simulink model "ECO_RM_WEC_SD_PI"  (R2025a)
settings: Solver=ode4  StartTime=0  StopTime=120  FixedStep=0.00025  MaxStep=0.00025  RelTol=1e-3
values from neighbouring files (symbols this model uses):
  s = tf('s')    [Compensated_loop_analysis.m]    (also in Plant_analysis.m)
  simu = simulationClass()    [wecSimInputFile.m]
  Z = (B + Bv)      + 1i*(omega0*(M + A) - C/omega0)    [Reference_velocity_calculation.m]
undefined symbols (not defined in the file or in its folder): body, constraint, geometry, hydroData, pto, X, Y
libraries: nesl_utility x9, sm_lib x5, WECSim_Lib_Body_Elements x2, WECSim_Lib_Frames x1, slpidlib x1, WECSim_Lib_Constraints x1
settings Model: Creator=pam1061  LastModifiedBy=Viki Vagnerova
settings SolverCC: ZeroCrossControl=DisableAll  AutoInsertRateTranBlk=on
settings DataIOCC: ReturnWorkspaceOutputs=off
settings OptimizationCC: SimCompilerOptimization=on

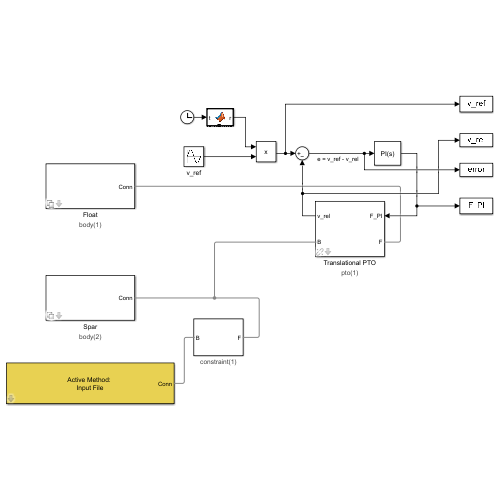
[thumbnail: Simulink's stored preview of the top-level diagram]
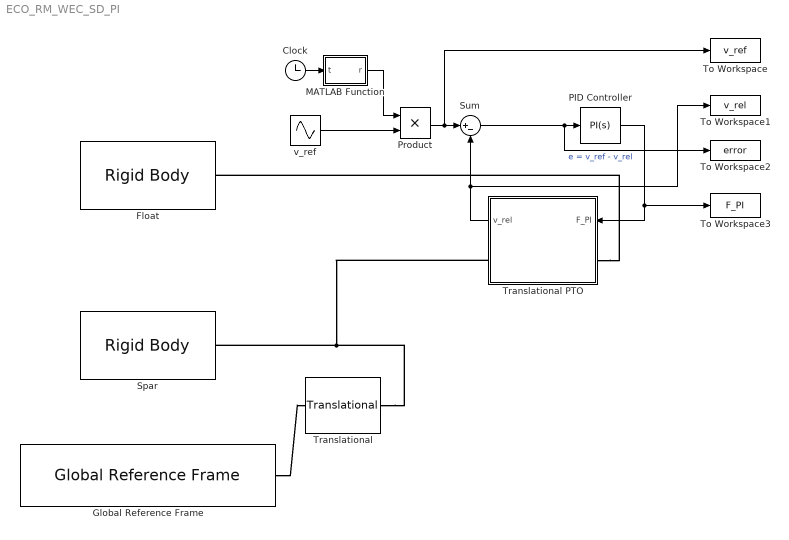
== system ECO_RM_WEC_SD_PI ==
  Clock : Clock
  Float : WECSim_Lib_Body_Elements/Rigid Body  body=body(1)  h5File=hydroData/*.h5  geometryFile=geometry/*.stl  mass=0  inertia=0 0 0  inertiaProducts=0 0 0  nonHydro=0  nonlinearHydro=0  centerGravity=0 0 0  centerBuoyancy=0 0 0  dof=6  volume=0  displacement=0 0 0  axis=0 1 0  angle=0  option=0  cd=0 0 0  ca=0 0 0  area=0 0 0  VME=0  rgME=0 0 0  z=0 0 1
  Global Reference Frame : WECSim_Lib_Frames/Global Reference Frame  waves=waves  simu=simu  InputMethod=Input File  InputFile=wecSimInputFile.m  mode=normal  explorer=off  solver=ode4  startTime=0  rampTime=100  endTime=400  dt=0.1  cicEndTime=60  stateSpace=0  WaveClass=regular  height=2.5  period=8  elevationFile=NOT DEFINED  spectrumFile=NOT DEFINED  direction=0  spread=1  spectrumType=NOT DEFINED  phaseSeed=0  option=EqualEnergy
  MATLAB Function : MATLAB Function  TreatAsAtomicUnit=on
  PID Controller : slpidlib/PID Controller  Controller=PI  Form=Parallel  TimeDomain=Continuous-time  UseExternalTs=off  SampleTime=-1  IntegratorMethod=Forward Euler  FilterMethod=Forward Euler  ControllerParametersSource=internal  P=1625.088066  I=4991.194750  UseKiTs=off  D=0  UseExternalDerivativeSource=off  N=100  UseFilter=on  TunerSelectOption=Transfer Function Based (PID Tuner App)  InitialConditionSource=internal  InitialConditionForIntegrator=0  InitialConditionForFilter=0  DifferentiatorICPrevScaledInput=0  ExternalReset=none  TrackingMode=off  Kt=1  LimitOutput=off  SatLimitsSource=internal  UpperSaturationLimit=inf  LowerSaturationLimit=-inf  LinearizeAsGain=on  AntiWindupMode=none  Kb=1  LimitIntegrator=off  UpperIntegratorSaturationLimit=inf  LowerIntegratorSaturationLimit=-inf  POutMin=[]  POutMax=[]  IOutMin=[]  IOutMax=[]  DOutMin=[]  DOutMax=[]  NOutMin=[]  NOutMax=[]  SumOutMin=[]  SumOutMax=[]  SaturationOutMin=[]  SaturationOutMax=[]  PParamMin=[]  PParamMax=[]  IParamMin=[]  IParamMax=[]  DParamMin=[]  DParamMax=[]  NParamMin=[]  NParamMax=[]  KbParamMin=[]  KbParamMax=[]  KtParamMin=[]  KtParamMax=[]  KbOutMin=[]  KbOutMax=[]  KtOutMin=[]  KtOutMax=[]  IntegratorOutMin=[]  IntegratorOutMax=[]  FilterOutMin=[]  FilterOutMax=[]  SumI1OutMin=[]  SumI1OutMax=[]  SumI2OutMin=[]  SumI2OutMax=[]  SumI3OutMin=[]  SumI3OutMax=[]  SumI4OutMin=[]  SumI4OutMax=[]  SumDOutMin=[]  SumDOutMax=[]  DifferentiatorOutMin=[]  DifferentiatorOutMax=[]  FilterDiffOutCoefMin=[]  FilterDiffOutCoefMax=[]  ReciprocalOutMin=[]  ReciprocalOutMax=[]  SumDenOutMin=[]  SumDenOutMax=[]  SumNumOutMin=[]  SumNumOutMax=[]  DivideOutMin=[]  DivideOutMax=[]  UdiffTsProdOutMin=[]  UdiffTsProdOutMax=[]  NTsProdOutMin=[]  NTsProdOutMax=[]  UintegralTsProdOutMin=[]  UintegralTsProdOutMax=[]  UngainTsProdOutMin=[]  UngainTsProdOutMax=[]  ClampingZeroOutDataTypeStr=Inherit: Inherit via back propagation  ClampingZeroOutMin=[]  ClampingZeroOutMax=[]  FilterDenConstantOutDataTypeStr=Inherit: Inherit via back propagation  FilterDenConstantOutMin=[]  FilterDenConstantOutMax=[]  PCopyOutDataTypeStr=Inherit: Inherit via back propagation  PCopyOutMin=[]  PCopyOutMax=[]  NCopyOutDataTypeStr=Inherit: Inherit via back propagation  NCopyOutMin=[]  NCopyOutMax=[]  IntegratorContinuousStateAttributes=''  IntegratorStateMustResolveToSignalObject=off  IntegratorRTWStateStorageClass=Auto  FilterContinuousStateAttributes=''  FilterStateMustResolveToSignalObject=off  FilterRTWStateStorageClass=Auto  ParallelPVariant=InternalParameters  IdealPVariant=Disabled  IVariant=InternalParameters  DVariant=Disabled  IntegratorVariant=Continuous  SatVariant=Disabled  AWVariant=Passthrough  PCopyVariant=Disabled  TRVariant=Disabled  FdbkBlocksVariant=Forward  IdealPFdbkVariant=Disabled  SatFdbkVariant=Disabled  DerivativeFilterVariant=Disabled  NVariant=Disabled  NCopyVariant=Disabled_SignalSpec  FilterICVariant=Disabled  IntegratorICVariant=InternalICs  ExternalResetVariant=Disabled  TRSumVariant=Passthrough  SumFdbkVariant=Disabled  SumVariant=Sum_PI  TsampFilterVariant=InternalTs  TsampNgainVariant=Passthrough  TsampIntegralVariant=Disabled_SignalSpec  ExternalSaturationOutDataTypeStr=Inherit: Same as second input  DerivativeSourceVariant=Disabled  PreIntVariant=InternalPreInt
  Product : Product
  Spar : WECSim_Lib_Body_Elements/Rigid Body  body=body(2)  h5File=hydroData/*.h5  geometryFile=geometry/*.stl  mass=0  inertia=0 0 0  inertiaProducts=0 0 0  nonHydro=0  nonlinearHydro=0  centerGravity=0 0 0  centerBuoyancy=0 0 0  dof=6  volume=0  displacement=0 0 0  axis=0 1 0  angle=0  option=0  cd=0 0 0  ca=0 0 0  area=0 0 0  VME=0  rgME=0 0 0  z=0 0 1
  Sum : Sum  Inputs=|+-
  To Workspace : ToWorkspace  VariableName=v_ref  SaveFormat=Timeseries  SampleTime=-1
  To Workspace1 : ToWorkspace  VariableName=v_rel  SaveFormat=Timeseries  SampleTime=-1
  To Workspace2 : ToWorkspace  VariableName=error  SaveFormat=Timeseries  SampleTime=-1
  To Workspace3 : ToWorkspace  VariableName=F_PI  SaveFormat=Timeseries  SampleTime=-1
  Translational : WECSim_Lib_Constraints/Translational  constraint=constraint(1)  loc="0  0  0"  displacement=0 0 0  y=0 1 0  z=0 0 1  upperLimitSpecify=off  upperLimitBound=0  upperLimitTransitionRegionWidth=0  upperLimitStiffness=0  upperLimitDamping=0  lowerLimitSpecify=off  lowerLimitBound=0  lowerLimitTransitionRegionWidth=0  lowerLimitStiffness=0  lowerLimitDamping=0
      settings: AttributesFormatString=%<constraint>
  Translational PTO : Subsystem  AncestorBlock=WECSim_Lib_PTOs/Translational PTO  mask(PTO){pto=pto(1), InputFileText=Global Reference Frame option "Use Input File" is selected., loc=0  0  0, stiffness=0, damping=0, equilibriumPosition=0, pretension=0, displacement=0 0 0, x=, y=0 1 0, z=0 0 1, upperLimitSpecify=off, upperLimitBound=0, upperLimitTransitionRegionWidth=0, upperLimitStiffness=0, upperLimitDamping=0, lowerLimitSpecify=off, lowerLimitBound=0, lowerLimitTransitionRegionWidth=0, lowerLimitStiffness=0, lowerLimitDamping=0}
      mask prompts: pto "PTO Name:"; loc "Location [m]:"; stiffness "Stiffness [N/m]:"; damping "Damping [N/(m/s)]:"; equilibriumPosition "Equilibrium position [m, deg]:"; pretension "Pretension [N, Nm]:"; displacement "Initial linear displacement [m]:"; x "X-axis [m]:"; y "Y-axis [m]:"; z "Z-axis [m]:"; upperLimitSpecify "Upper limit"; upperLimitBound "Upper limit bound [m, deg]:"; upperLimitTransitionRegionWidth "Upper limit transition region width [m, deg]:"; upperLimitStiffness "Upper limit stiffness [N/m, Nm/rad]:"; upperLimitDamping "Upper limit damping [N/(m/s), Nm/(rad/s)]:"; lowerLimitSpecify "Lower limit"; lowerLimitBound "Upper limit bound [m, deg]:"; lowerLimitTransitionRegionWidth "Upper limit transition region width [m, deg]:"; lowerLimitStiffness "Upper limit stiffness [N/m, Nm/rad]:"; lowerLimitDamping "Upper limit damping [N/(m/s), Nm/(rad/s)]:"
      mask help:
      | Constrains the follower to translational motion relative to the base, in
      | the PTO's Z-direction and adds PTO stiffness and damping.
      |
      |
      | The variable name input below must be 'pto(i)' where i=1,2,...
      | pto(i) must be defined in the input file with the following fields:
      |
      |     .name (required)
      |             String.
      |             PTO name. Must comply with Matlab's variable naming rules.
      |     .location (optional)
      |             3x1 vector [x y z] in meters.
      |             PTO location. Default = [0 0 0]
      |     .stiffness (optional)
      |             Float.
      |             PTO linear spring stiffness. Default = 0
      |     .damping (optional)
      |             Float.
      |             PTO linear damping coefficient. Default = 0
      |     .orientation.z (optional)
      |             3x1 vector [x y z].
      |             Direction of the PTO's Z-coordinate. Default = [0 0 1]
      |     .orientation.y (optional)
      |             3x1 vector [x y z].
      |             Direction of the PTO's Y-coordinate. Default = [0 1 0]
      mask init:
      | if exist('pto','var')
      |     h=[gcb '/To Workspace'];
      |     responseName=['pto' num2str(pto.number) '_out'];
      |     set_param(h,'VariableName',responseName);
      |     h=[gcb '/Translational PCC' newline '(Prismatic Joint)'];
      |     try % this should catch any version issue for which these parameters do not exist
      |         set_param(h,'upperLimitSpecify',pto.hardStops.upperLimitSpecify)
      |         set_param(h,'lowerLimitSpecify',pto.hardStops.lowerLimitSpecify)
      |     end
      | end
      | 
      | pto.checkLoc('W');
      settings: AttributesFormatString=%<pto>
      mask Help:
      | Constrains the follower to translational motion relative to the base, in
      | the PTO's Z-direction and adds PTO stiffness and damping.
      | 
      | 
      | The variable name input below must be 'pto(i)' where i=1,2,...
      | pto(i) must be defined in the input file with the following fields:
      | 
      |     .name (required)
      |             String.
      |             PTO name. Must comply with Matlab's variable naming rules.
      |     .location (optional)
      |             3x1 vector [x y z] in meters.
      |             PTO location. Default = [0 0 0]
      |     .stiffness (optional)
      |             Float.
      |             PTO linear spring stiffness. Default = 0
      |     .damping (optional)
      |             Float.
      |             PTO linear damping coefficient. Default = 0
      |     .orientation.z (optional)
      |             3x1 vector [x y z].
      |             Direction of the PTO's Z-coordinate. Default = [0 0 1]
      |     .orientation.y (optional)
      |             3x1 vector [x y z].
      |             Direction of the PTO's Y-coordinate. Default = [0 1 0]
      mask Callback upperLimitSpecify: hardStopCallback(gcbh)
      mask Callback lowerLimitSpecify: hardStopCallback(gcbh)
      mask DialogControl InputFileGroup Prompt: Input File
      mask DialogControl CustomParameterGroup Prompt: Custom Parameters
      mask DialogControl std_opts Prompt: Standard options
      mask DialogControl orientations Prompt: Orientation
      mask DialogControl x Tooltip: This axis is defined by the y and z axes.
      mask DialogControl Container7 Prompt: Hard Stop
  v_ref : Sin  Amplitude=1.039494  Frequency=4  Phase=1.94184  SampleTime=0
  wires:
  Translational PTO/1(v_rel) -> To Workspace1/1, Sum/2
  Sum/1 -> To Workspace2/1, PID Controller/1  "e = v_ref - v_rel"
  PID Controller/1 -> Translational PTO/1(F_PI), To Workspace3/1
  Clock/1 -> MATLAB Function/1(t)
  Product/1 -> To Workspace/1, Sum/1
  v_ref/1 -> Product/2
  MATLAB Function/1(r) -> Product/1
  connections:
  Global Reference Frame/RConn1 -- Translational/LConn1
  Translational/RConn1 -- Translational PTO/RConn1 -- Spar/RConn1
  Translational PTO/LConn1 -- Float/RConn1

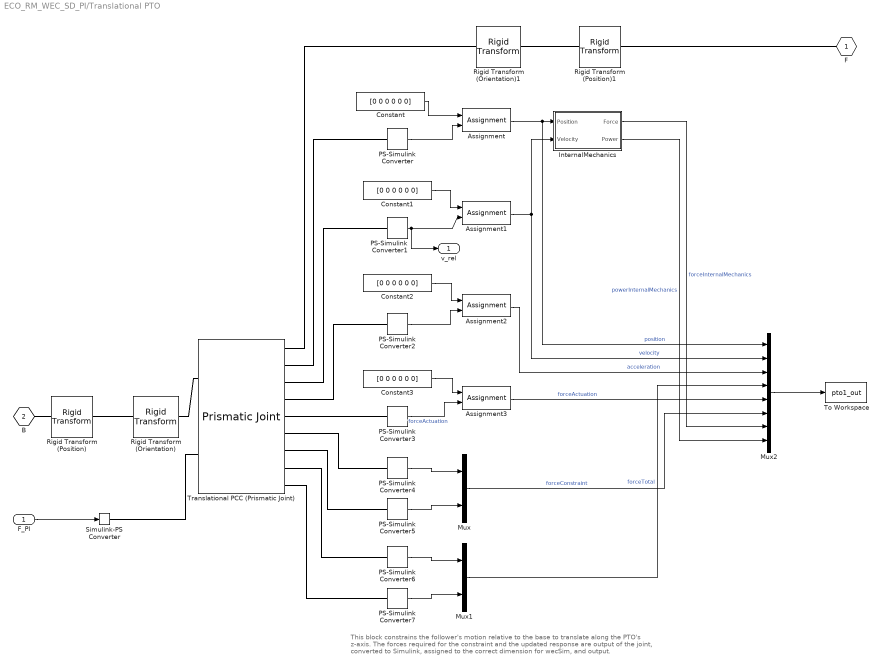
== system ECO_RM_WEC_SD_PI/Translational PTO ==
  note: This block constrains the follower's motion relative to the base to translate along the PTO's z-axis. The forces required for the constraint and the updated response are output of the joint, converted to Simulink, assigned to the correct dimension for wecSim, and output.
  F_PI : Inport
  Assignment{,1..3} (4 alike) : Assignment  IndexOptions=Index vector (dialog)  Indices=3  OutputSizes=1
  Constant{,1..3} (4 alike) : Constant  Value=[0 0 0 0 0 0]
  InternalMechanics : Subsystem
  Mux : Mux  Inputs=2
  Mux1 : Mux  Inputs=2
  Mux2 : Mux  Inputs=8
  PS-Simulink Converter{,1..7} (8 alike) : nesl_utility/PS-Simulink Converter  PhysicalDomain=network_engine_domain  SubClassName=ps_output  LeftPortType=input  RightPortType=output  PseudoPeriodic=off  Frequencies=[]  VectorFormat=1-D array  Unit=1  AffineConversion=off
  Rigid Transform (Position) : sm_lib/Frames and Transforms/Rigid Transform  RotationMethod=None  FollAlignAxisA=+X  BaseAlignAxisA=+Y  FollAlignAxisB=+Y  BaseAlignAxisB=+Z  RotationStandardAxis=+Y  RotationAngle=0  RotationAngleUnits=rad  RotationArbitraryAxis=[0 1 0]  RotationSequenceAxes=FollowerAxes  RotationSequence=XYX  RotationSequenceAngles=[0 0 0]  RotationSequenceAnglesUnits=deg  RotationMatrix=[1 0 0; 0 1 0; 0 0 1]  Quaternion=[1 0 0 0]  TranslationMethod=Cartesian  TranslationCartesianOffset=pto.initial.displacement + pto.location  TranslationCartesianOffsetUnits=m  TranslationStandardAxis=+Z  TranslationStandardOffset=0  TranslationStandardOffsetUnits=m  TranslationROffset=0  TranslationROffsetUnits=m  TranslationThetaOffset=0  TranslationThetaOffsetUnits=deg  TranslationZOffset=0  TranslationZOffsetUnits=m
  Rigid Transform (Position)1 : sm_lib/Frames and Transforms/Rigid Transform  RotationMethod=None  FollAlignAxisA=+X  BaseAlignAxisA=+Y  FollAlignAxisB=+Y  BaseAlignAxisB=+Z  RotationStandardAxis=+Y  RotationAngle=0  RotationAngleUnits=rad  RotationArbitraryAxis=[0 1 0]  RotationSequenceAxes=FollowerAxes  RotationSequence=XYX  RotationSequenceAngles=[0 0 0]  RotationSequenceAnglesUnits=deg  RotationMatrix=[1 0 0; 0 1 0; 0 0 1]  Quaternion=[1 0 0 0]  TranslationMethod=Cartesian  TranslationCartesianOffset=pto.initial.displacement + pto.location  TranslationCartesianOffsetUnits=m  TranslationStandardAxis=+Z  TranslationStandardOffset=0  TranslationStandardOffsetUnits=m  TranslationROffset=0  TranslationROffsetUnits=m  TranslationThetaOffset=0  TranslationThetaOffsetUnits=deg  TranslationZOffset=0  TranslationZOffsetUnits=m
  Rigid Transform (Orientation) : sm_lib/Frames and Transforms/Rigid Transform  RotationMethod=RotationMatrix  FollAlignAxisA=+X  BaseAlignAxisA=+Y  FollAlignAxisB=+Y  BaseAlignAxisB=+Z  RotationStandardAxis=+Y  RotationAngle=0  RotationAngleUnits=rad  RotationArbitraryAxis=[0 1 0]  RotationSequenceAxes=FollowerAxes  RotationSequence=XYX  RotationSequenceAngles=[0 0 0]  RotationSequenceAnglesUnits=deg  RotationMatrix=pto.orientation.rotationMatrix  Quaternion=[1 0 0 0]  TranslationMethod=None  TranslationCartesianOffset=0  TranslationCartesianOffsetUnits=m  TranslationStandardAxis=+Z  TranslationStandardOffset=0  TranslationStandardOffsetUnits=m  TranslationROffset=0  TranslationROffsetUnits=m  TranslationThetaOffset=0  TranslationThetaOffsetUnits=deg  TranslationZOffset=0  TranslationZOffsetUnits=m
  Rigid Transform (Orientation)1 : sm_lib/Frames and Transforms/Rigid Transform  RotationMethod=RotationMatrix  FollAlignAxisA=+X  BaseAlignAxisA=+Y  FollAlignAxisB=+Y  BaseAlignAxisB=+Z  RotationStandardAxis=+Y  RotationAngle=0  RotationAngleUnits=rad  RotationArbitraryAxis=[0 1 0]  RotationSequenceAxes=FollowerAxes  RotationSequence=XYX  RotationSequenceAngles=[0 0 0]  RotationSequenceAnglesUnits=deg  RotationMatrix=pto.orientation.rotationMatrix  Quaternion=[1 0 0 0]  TranslationMethod=None  TranslationCartesianOffset=0  TranslationCartesianOffsetUnits=m  TranslationStandardAxis=+Z  TranslationStandardOffset=0  TranslationStandardOffsetUnits=m  TranslationROffset=0  TranslationROffsetUnits=m  TranslationThetaOffset=0  TranslationThetaOffsetUnits=deg  TranslationZOffset=0  TranslationZOffsetUnits=m
  Simulink-PS Converter : nesl_utility/Simulink-PS Converter  PhysicalDomain=network_engine_domain  SubClassName=ps_input  LeftPortType=input  RightPortType=output  PseudoPeriodic=off  Frequencies=[]  NoiseDistribution=none  NoiseParameters=[]  Unit=N  AffineConversion=off  FilteringAndDerivatives=provide  SimscapeFilterOrder=1  InputFilterTimeConstant=0.001  UdotUserProvided=0
  To Workspace : ToWorkspace  VariableName=pto1_out  SaveFormat=Structure With Time  SampleTime=simu.dtOut
  Translational PCC (Prismatic Joint) : sm_lib/Joints/Prismatic Joint  JointMode=Normal  CompositeWrenchDir=BaseOnFollower  CompositeWrenchFrame=BaseFrame  SenseConstraintForce=on  SenseConstraintTorque=on  SenseTotalForce=on  SenseTotalTorque=on  PositionTargetSpecify=off  PositionTargetPriority=High  PositionTargetValue=0  PositionTargetValueUnits=m  VelocityTargetSpecify=off  VelocityTargetPriority=High  VelocityTargetValue=0  VelocityTargetValueUnits=m/s  EquilibriumPosition=pto.equilibriumPosition  EquilibriumPositionUnits=m  SpringStiffness=pto.stiffness  SpringStiffnessUnits=N/m  DampingCoefficient=pto.damping  DampingCoefficientUnits=N/(m/s)  LowerLimitSpecify=off  LowerLimitBound=pto.hardStops.lowerLimitBound  LowerLimitBoundUnits=m  LowerLimitStiffness=pto.hardStops.lowerLimitStiffness  LowerLimitStiffnessUnits=N/m  LowerLimitDamping=pto.hardStops.lowerLimitDamping  LowerLimitDampingUnits=N/(m/s)  LowerLimitTransitionRegionWidth=pto.hardStops.lowerLimitTransitionRegionWidth  LowerLimitTransitionRegionWidthUnits=m  UpperLimitSpecify=off  UpperLimitBound=pto.hardStops.upperLimitBound  UpperLimitBoundUnits=m  UpperLimitStiffness=pto.hardStops.upperLimitStiffness  UpperLimitStiffnessUnits=N/m  UpperLimitDamping=pto.hardStops.upperLimitDamping  UpperLimitDampingUnits=N/(m/s)  UpperLimitTransitionRegionWidth=pto.hardStops.upperLimitTransitionRegionWidth  UpperLimitTransitionRegionWidthUnits=m  TorqueActuationMode=InputTorque  MotionActuationMode=ComputedMotion  SensePosition=on  SenseVelocity=on  SenseAcceleration=on  SenseTorqueForce=on  SenseLowerLimitTorqueForce=off  SenseUpperLimitTorqueForce=off
  F : PMIOPort  Side=Left
  B : PMIOPort  Port=2  Side=Right
  v_rel : Outport
  wires:
  Mux2/1 -> To Workspace/1
  Mux/1 -> Mux2/6  "forceConstraint"
  Mux1/1 -> Mux2/4  "forceTotal"
  PS-Simulink Converter4/1 -> Mux/1
  PS-Simulink Converter5/1 -> Mux/2
  PS-Simulink Converter6/1 -> Mux1/1
  PS-Simulink Converter7/1 -> Mux1/2
  Assignment3/1 -> Mux2/5  "forceActuation"
  Assignment/1 -> Mux2/1, InternalMechanics/1(Position)  "position"
  Assignment1/1 -> Mux2/2, InternalMechanics/2(Velocity)  "velocity"
  Assignment2/1 -> Mux2/3  "acceleration"
  Constant/1 -> Assignment/1
  PS-Simulink Converter/1 -> Assignment/2
  Constant1/1 -> Assignment1/1
  Constant2/1 -> Assignment2/1
  PS-Simulink Converter2/1 -> Assignment2/2
  InternalMechanics/1(Force) -> Mux2/7  "forceInternalMechanics"
  InternalMechanics/2(Power) -> Mux2/8  "powerInternalMechanics"
  Constant3/1 -> Assignment3/1
  PS-Simulink Converter3/1 -> Assignment3/2  "forceActuation"
  F_PI/1 -> Simulink-PS Converter/1
  PS-Simulink Converter1/1 -> v_rel/1, Assignment1/2
  connections:
  Rigid Transform (Position)/LConn1 -- B/RConn1
  Translational PCC (Prismatic Joint)/RConn5 -- PS-Simulink Converter3/LConn1
  Translational PCC (Prismatic Joint)/RConn9 -- PS-Simulink Converter7/LConn1
  Rigid Transform (Orientation)1/RConn1 -- Translational PCC (Prismatic Joint)/RConn1
  Translational PCC (Prismatic Joint)/RConn4 -- PS-Simulink Converter2/LConn1
  Translational PCC (Prismatic Joint)/RConn7 -- PS-Simulink Converter5/LConn1
  Translational PCC (Prismatic Joint)/RConn3 -- PS-Simulink Converter1/LConn1
  Rigid Transform (Position)1/LConn1 -- F/RConn1
  Translational PCC (Prismatic Joint)/RConn8 -- PS-Simulink Converter6/LConn1
  Translational PCC (Prismatic Joint)/RConn2 -- PS-Simulink Converter/LConn1
  Translational PCC (Prismatic Joint)/RConn6 -- PS-Simulink Converter4/LConn1
  Rigid Transform (Orientation)/RConn1 -- Translational PCC (Prismatic Joint)/LConn1
  Rigid Transform (Position)1/RConn1 -- Rigid Transform (Orientation)1/LConn1
  Rigid Transform (Position)/RConn1 -- Rigid Transform (Orientation)/LConn1
  Simulink-PS Converter/RConn1 -- Translational PCC (Prismatic Joint)/LConn2

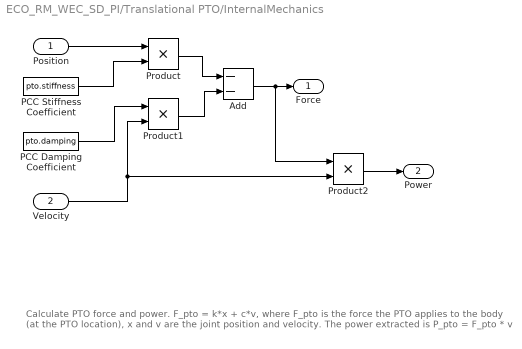
== system ECO_RM_WEC_SD_PI/Translational PTO/InternalMechanics ==
  note: Calculate PTO force and power.
      |
      | F_pto  = k*x + c*v,
      | where F_pto is the force the PTO applies to the body (at the PTO location), x and v are the joint position and velocity.
      |
      | The power extracted is
      | P_pto = F_pto * v
  Position : Inport
  Velocity : Inport  Port=2
  Add : Sum  Inputs=--
  PCC Damping Coefficient : Constant  Value=pto.damping
  PCC Stiffness Coefficient : Constant  Value=pto.stiffness
  Product : Product  Inputs=**
  Product1 : Product  Inputs=**
  Product2 : Product  Inputs=**
  Force : Outport
  Power : Outport  Port=2
  wires:
  PCC Damping Coefficient/1 -> Product1/1
  Product2/1 -> Power/1
  PCC Stiffness Coefficient/1 -> Product/2
  Position/1 -> Product/1
  Add/1 -> Product2/1, Force/1
  Velocity/1 -> Product2/2, Product1/2
  Product/1 -> Add/1
  Product1/1 -> Add/2

== matlab function ECO_RM_WEC_SD_PI/MATLAB Function ==
  data: t input; r output
function r = wecRamp(t)

Tr = 30;

if t < Tr
    r = 0.5*(1 - cos(pi*t/Tr));
else
    r = 1;
end
